simulink model "ASM_Traffic"  (R2026a)
settings: Solver=ode1  StartTime=SIM.tstart.v  StopTime=SIM.tend.v  FixedStep=SIM.StepSize.v
PostLoadFcn:
  | if any(exist('dsrtsu_mdlpostloadfcn', 'file') ~= 0), dsrtsu_mdlpostloadfcn('Execute', bdroot); end
  | try, asm_mdl_postloadfcn(bdroot, 'UpdateModel', 3600); catch, disp(lasterr); end,
InitFcn:
  | , if any(exist('rtifpga_mdlclblib', 'file') ~= 0), rtifpga_mdlclblib('Init', bdroot); end,
  | , if any(exist('dsmpb_private', 'file') ~= 0), dsmpb_private('dsmpb_mdlclblib', 'Init', bdroot); end,
model workspace (MAT data in the model file):
  asmReferencePath = [0 0.01 0.02 0.03 0.04 0.05 0.06 0.07 0.08 0.09 0.1 0.11 ... (350007 elements, 50001x7)]
  roadBounds : Simulink.Parameter (value not decoded)
  safetyAxes : Simulink.Parameter (value not decoded)
undefined symbols (not defined in the file): _to_, a0b2, ASM_BrakeHydraulics_DemoSystems, ASM_VehicleDynamics_DemoSystems, b98103fe8ad365046cd0, BrakeCircuit, controllerConfig, CPT, Crankshaft, DiscIntNeverNeededParam, dsmsi, FinalDriveAssembly, MDL, ModeSignals, mu, Pos_BrakePedal_Maneuver, rad, RefSignals, roadFamilyData, roadFamilyId, s_to_rpm, SIM, SoftECU, Suspension, Tire, Transmission
libraries: ASM_Traffic_lib x135, simulink x98, ASM_Utils_lib x77, ASM_VehicleDynamics_lib x70, ASM_Environment_lib x22, dsmpblib x20, dsmsilib x15, MDLD_Utils_lib x10, ASM_BrakeHydraulics_lib x3, sl_discontinuities x2
(part 38 of 65)

== system ASM_Traffic/Engine/Plant/UserInterface/DISP_Plant/Fuel_Consumption[L|100km]_ ==
  note: If v_Vehicle < v_Vehicle_LowLim, Then FuelConsumption = [L|h]
      | Else, FuelConsumption = [L|100km]
  v_Vehicle[km|h] : Inport
  Fuel_Consumption[l|h] : Inport  Port=2
  100 : Constant  Value=100
  999 : Constant  Value=999
  FuelConsumption : Terminator
  FuelConsumption[L|100km]_ : Product  Inputs=/**  SaturateOnIntegerOverflow=on  OutDataTypeStr=Inherit: Same as first input
  Sat_v_Vehicle[km|h] : Saturate  UpperLimit=inf  LowerLimit=eps
  Sw_FuelConsumption[L|100km] : MultiPortSwitch  DataPortOrder=Zero-based contiguous  Inputs=2  zeroidx=on  SaturateOnIntegerOverflow=off  InputSameDT=off
  Sw_[L|100km]2[L|h] : Switch  Criteria=u2 > Threshold  SaturateOnIntegerOverflow=off  InputSameDT=off
  v_Vehicle_LowLim[km|h] : simulink/Logic and Bit Operations/Compare To Constant  relop=>=  const=1  OutDataTypeStr=boolean
  Fuel_Consumption[L|100km] : Outport  VectorParamsAs1DForOutWhenUnconnected=off
  wires:
  999/1 -> Sw_FuelConsumption[L|100km]/2
  FuelConsumption[L|100km]_/1 -> Sw_FuelConsumption[L|100km]/3
  Sw_[L|100km]2[L|h]/1 -> FuelConsumption/1
  v_Vehicle_LowLim[km|h]/1 -> Sw_[L|100km]2[L|h]/2, Sw_FuelConsumption[L|100km]/1
  Sat_v_Vehicle[km|h]/1 -> FuelConsumption[L|100km]_/1
  100/1 -> FuelConsumption[L|100km]_/3
  Fuel_Consumption[l|h]/1 -> Sw_[L|100km]2[L|h]/3, FuelConsumption[L|100km]_/2
  v_Vehicle[km|h]/1 -> v_Vehicle_LowLim[km|h]/1, Sat_v_Vehicle[km|h]/1
  Sw_FuelConsumption[L|100km]/1 -> Sw_[L|100km]2[L|h]/1, Fuel_Consumption[L|100km]/1

== system ASM_Traffic/Engine/Plant/UserInterface/DISP_Plant/Fuel_Consumption[l|h] ==
  In1 : Inport
  Out1 : Outport  VectorParamsAs1DForOutWhenUnconnected=off
  wires:
  In1/1 -> Out1/1

== system ASM_Traffic/Engine/Plant/UserInterface/DISP_Plant/Fuel_Consumption_Total[l] ==
  In1 : Inport
  Out1 : Outport  VectorParamsAs1DForOutWhenUnconnected=off
  wires:
  In1/1 -> Out1/1

== system ASM_Traffic/Engine/Plant/UserInterface/DISP_Plant/T_Water[degC] ==
  In1 : Inport
  Out1 : Outport  VectorParamsAs1DForOutWhenUnconnected=off
  wires:
  In1/1 -> Out1/1

== system ASM_Traffic/Engine/Plant/UserInterface/DISP_Plant/Trq_Eff_Engine[Nm] ==
  In1 : Inport
  Out1 : Outport  VectorParamsAs1DForOutWhenUnconnected=off
  wires:
  In1/1 -> Out1/1

== system ASM_Traffic/Engine/Plant/UserInterface/DISP_Plant/Trq_Fric_Engine[Nm] ==
  In1 : Inport
  Out1 : Outport  VectorParamsAs1DForOutWhenUnconnected=off
  wires:
  In1/1 -> Out1/1

== system ASM_Traffic/Engine/Plant/UserInterface/DISP_Plant/Trq_Ind_Engine[Nm] ==
  In1 : Inport
  Out1 : Outport  VectorParamsAs1DForOutWhenUnconnected=off
  wires:
  In1/1 -> Out1/1

== system ASM_Traffic/Engine/Plant/UserInterface/DISP_Plant/b_e[g|kWh] ==
  In1 : Inport
  Out1 : Outport  VectorParamsAs1DForOutWhenUnconnected=off
  wires:
  In1/1 -> Out1/1

== system ASM_Traffic/Engine/Plant/UserInterface/DISP_Plant/eta_Eff_Engine[0_1] ==
  In1 : Inport
  Out1 : Outport  VectorParamsAs1DForOutWhenUnconnected=off
  wires:
  In1/1 -> Out1/1

== system ASM_Traffic/Engine/Plant/UserInterface/DISP_Plant/eta_Ind_Engine[0_1] ==
  In1 : Inport
  Out1 : Outport  VectorParamsAs1DForOutWhenUnconnected=off
  wires:
  In1/1 -> Out1/1

== system ASM_Traffic/Engine/Plant/UserInterface/DISP_Plant/eta_Mechanical_Engine[0_1] ==
  In1 : Inport
  Out1 : Outport  VectorParamsAs1DForOutWhenUnconnected=off
  wires:
  In1/1 -> Out1/1

== system ASM_Traffic/Engine/Plant/UserInterface/DISP_Plant/mdot_Fuel[g|h] ==
  In1 : Inport
  Out1 : Outport  VectorParamsAs1DForOutWhenUnconnected=off
  wires:
  In1/1 -> Out1/1

== system ASM_Traffic/Engine/SignalInterface/ASMSignalInterface/signal_structure/InfoBlock ==

== system ASM_Traffic/Environment/GroundTruth/PlantModel/Add_Time/Reset_Time ==
  Seconds_In[s] : Inport
  Add5 : Sum  Inputs=+-
  Constant4 : Constant  Value=86400
  Constant5 : Constant  Value=86400
  Divide2 : Product  Inputs=*/
  Divide3 : Product  Inputs=**
  Rounding Function3 : Rounding
  Seconds_Out[s] : Outport  VectorParamsAs1DForOutWhenUnconnected=off
  wires:
  Divide3/1 -> Add5/2
  Divide2/1 -> Rounding Function3/1
  Constant5/1 -> Divide3/2
  Add5/1 -> Seconds_Out[s]/1
  Seconds_In[s]/1 -> Add5/1, Divide2/1
  Constant4/1 -> Divide2/2
  Rounding Function3/1 -> Divide3/1

== system ASM_Traffic/Environment/GroundTruth/PlantModel/GroundTruth_Data_Access/GroundTruth_Access_Laneboundaries ==
  Enable[0Off|1On] : Inport
  OSI_GT_Data : Inport  Port=2
  Enable : EnablePort
  asm_trf_osi_access_laneboundaries : S-Function  FunctionName=asm_trf_osi_access_laneboundaries  Parameters=10,15  SFunctionDeploymentMode=off  EnableBusSupport=off
  Num_Laneboundaries[] : Outport  VectorParamsAs1DForOutWhenUnconnected=off
  Laneboundary_ID[] : Outport  Port=2  VectorParamsAs1DForOutWhenUnconnected=off
  Laneboundary_Type[] : Outport  Port=3  VectorParamsAs1DForOutWhenUnconnected=off
  Laneboundary_Color[] : Outport  Port=4  VectorParamsAs1DForOutWhenUnconnected=off
  Num_Laneboundary_Points[] : Outport  Port=5  VectorParamsAs1DForOutWhenUnconnected=off
  Laneboundary_Point_Width[m] : Outport  Port=6  VectorParamsAs1DForOutWhenUnconnected=off
  Laneboundary_Point_Height[m] : Outport  Port=7  VectorParamsAs1DForOutWhenUnconnected=off
  Laneboundary_Point_Pos_x[m] : Outport  Port=8  VectorParamsAs1DForOutWhenUnconnected=off
  Laneboundary_Point_Pos_y[m] : Outport  Port=9  VectorParamsAs1DForOutWhenUnconnected=off
  Laneboundary_Point_Pos_z[m] : Outport  Port=10  VectorParamsAs1DForOutWhenUnconnected=off
  Laneboundary_Point_Dash[] : Outport  Port=11  VectorParamsAs1DForOutWhenUnconnected=off
  wires:
  asm_trf_osi_access_laneboundaries/11 -> Laneboundary_Point_Dash[]/1
  asm_trf_osi_access_laneboundaries/10 -> Laneboundary_Point_Pos_z[m]/1
  asm_trf_osi_access_laneboundaries/9 -> Laneboundary_Point_Pos_y[m]/1
  asm_trf_osi_access_laneboundaries/8 -> Laneboundary_Point_Pos_x[m]/1
  asm_trf_osi_access_laneboundaries/7 -> Laneboundary_Point_Height[m]/1
  asm_trf_osi_access_laneboundaries/6 -> Laneboundary_Point_Width[m]/1
  asm_trf_osi_access_laneboundaries/5 -> Num_Laneboundary_Points[]/1
  asm_trf_osi_access_laneboundaries/4 -> Laneboundary_Color[]/1
  asm_trf_osi_access_laneboundaries/3 -> Laneboundary_Type[]/1
  asm_trf_osi_access_laneboundaries/2 -> Laneboundary_ID[]/1
  asm_trf_osi_access_laneboundaries/1 -> Num_Laneboundaries[]/1
  OSI_GT_Data/1 -> asm_trf_osi_access_laneboundaries/2
  Enable[0Off|1On]/1 -> asm_trf_osi_access_laneboundaries/1

== system ASM_Traffic/Environment/GroundTruth/PlantModel/GroundTruth_Data_Access/GroundTruth_Access_Lanes ==
  Enable[0Off|1On] : Inport
  OSI_GT_Data : Inport  Port=2
  asm_trf_osi_access_lanes : S-Function  FunctionName=asm_trf_osi_access_lanes  Parameters=20,10,10  SFunctionDeploymentMode=off  EnableBusSupport=off
  Num_Lanes[] : Outport  VectorParamsAs1DForOutWhenUnconnected=off
  Lane_ID[] : Outport  Port=2  VectorParamsAs1DForOutWhenUnconnected=off
  Lane_Type[] : Outport  Port=3  VectorParamsAs1DForOutWhenUnconnected=off
  Is_Host_Vehicle_Lane[0|1] : Outport  Port=4  VectorParamsAs1DForOutWhenUnconnected=off
  Num_Left_Adjacent_Lanes[] : Outport  Port=5  VectorParamsAs1DForOutWhenUnconnected=off
  Left_Adjacent_Lane_ID[m] : Outport  Port=6  VectorParamsAs1DForOutWhenUnconnected=off
  Num_Right_Adjacent_Lanes[] : Outport  Port=7  VectorParamsAs1DForOutWhenUnconnected=off
  Right_Adjacent_Lane_ID[m] : Outport  Port=8  VectorParamsAs1DForOutWhenUnconnected=off
  Num_Lane_Pairings[] : Outport  Port=9  VectorParamsAs1DForOutWhenUnconnected=off
  Successor_Lane_ID[] : Outport  Port=10  VectorParamsAs1DForOutWhenUnconnected=off
  Antecessor_Lane_ID[] : Outport  Port=11  VectorParamsAs1DForOutWhenUnconnected=off
  Num_Left_Laneboundaries[] : Outport  Port=12  VectorParamsAs1DForOutWhenUnconnected=off
  Left_Laneboundary_ID[] : Outport  Port=13  VectorParamsAs1DForOutWhenUnconnected=off
  Num_Right_Laneboundaries[] : Outport  Port=14  VectorParamsAs1DForOutWhenUnconnected=off
  Right_Laneboundary_ID[] : Outport  Port=15  VectorParamsAs1DForOutWhenUnconnected=off
  Num_Free_Laneboundaries[] : Outport  Port=16  VectorParamsAs1DForOutWhenUnconnected=off
  Free_Laneboundary_ID[] : Outport  Port=17  VectorParamsAs1DForOutWhenUnconnected=off
  wires:
  Enable[0Off|1On]/1 -> asm_trf_osi_access_lanes/1
  OSI_GT_Data/1 -> asm_trf_osi_access_lanes/2
  asm_trf_osi_access_lanes/1 -> Num_Lanes[]/1
  asm_trf_osi_access_lanes/2 -> Lane_ID[]/1
  asm_trf_osi_access_lanes/3 -> Lane_Type[]/1
  asm_trf_osi_access_lanes/4 -> Is_Host_Vehicle_Lane[0|1]/1
  asm_trf_osi_access_lanes/5 -> Num_Left_Adjacent_Lanes[]/1
  asm_trf_osi_access_lanes/6 -> Left_Adjacent_Lane_ID[m]/1
  asm_trf_osi_access_lanes/7 -> Num_Right_Adjacent_Lanes[]/1
  asm_trf_osi_access_lanes/8 -> Right_Adjacent_Lane_ID[m]/1
  asm_trf_osi_access_lanes/9 -> Num_Lane_Pairings[]/1
  asm_trf_osi_access_lanes/10 -> Successor_Lane_ID[]/1
  asm_trf_osi_access_lanes/11 -> Antecessor_Lane_ID[]/1
  asm_trf_osi_access_lanes/12 -> Num_Left_Laneboundaries[]/1
  asm_trf_osi_access_lanes/13 -> Left_Laneboundary_ID[]/1
  asm_trf_osi_access_lanes/14 -> Num_Right_Laneboundaries[]/1
  asm_trf_osi_access_lanes/15 -> Right_Laneboundary_ID[]/1
  asm_trf_osi_access_lanes/16 -> Num_Free_Laneboundaries[]/1
  asm_trf_osi_access_lanes/17 -> Free_Laneboundary_ID[]/1

== system ASM_Traffic/Environment/GroundTruth/PlantModel/GroundTruth_Data_Access/GroundTruth_Access_MovingObjects ==
  Enable[0Off|1On] : Inport
  Filter_MovObj_In_GT_Area[0Off|1On] : Inport  Port=2
  MovObj_Idx[] : Inport  Port=3
  OSI_GT_Data : Inport  Port=4
  asm_trf_osi_access_mov_obj : S-Function  FunctionName=asm_trf_osi_access_mov_obj  Parameters=10  SFunctionDeploymentMode=off  EnableBusSupport=off
  Num_MovObj[] : Outport  VectorParamsAs1DForOutWhenUnconnected=off
  Num_MovObj_in_GT_Area[] : Outport  Port=2  VectorParamsAs1DForOutWhenUnconnected=off
  Flag_MovObj_in_GT_Area[] : Outport  Port=3  VectorParamsAs1DForOutWhenUnconnected=off
  MovObj_Type[] : Outport  Port=4  VectorParamsAs1DForOutWhenUnconnected=off
  MovObj_Vehicle_Type[] : Outport  Port=5  VectorParamsAs1DForOutWhenUnconnected=off
  MovObj_ID[] : Outport  Port=6  VectorParamsAs1DForOutWhenUnconnected=off
  MovObj_Driver_ID[] : Outport  Port=7  VectorParamsAs1DForOutWhenUnconnected=off
  Flag_MovObj_HasTrailer[] : Outport  Port=8  VectorParamsAs1DForOutWhenUnconnected=off
  MovObj_Trailer_ID[] : Outport  Port=9  VectorParamsAs1DForOutWhenUnconnected=off
  MovObj_Position_x[m] : Outport  Port=10  VectorParamsAs1DForOutWhenUnconnected=off
  MovObj_Position_y[m] : Outport  Port=11  VectorParamsAs1DForOutWhenUnconnected=off
  MovObj_Position_z[m] : Outport  Port=12  VectorParamsAs1DForOutWhenUnconnected=off
  MovObj_Velocity_x[km|h] : Outport  Port=13  VectorParamsAs1DForOutWhenUnconnected=off
  MovObj_Velocity_y[km|h] : Outport  Port=14  VectorParamsAs1DForOutWhenUnconnected=off
  MovObj_Velocity_z[km|h] : Outport  Port=15  VectorParamsAs1DForOutWhenUnconnected=off
  MovObj_Acceleration_x[m|s2] : Outport  Port=16  VectorParamsAs1DForOutWhenUnconnected=off
  MovObj_Acceleration_y[m|s2] : Outport  Port=17  VectorParamsAs1DForOutWhenUnconnected=off
  MovObj_Acceleration_z[m|s2] : Outport  Port=18  VectorParamsAs1DForOutWhenUnconnected=off
  MovObj_Orientation_x[deg] : Outport  Port=19  VectorParamsAs1DForOutWhenUnconnected=off
  MovObj_Orientation_y[deg] : Outport  Port=20  VectorParamsAs1DForOutWhenUnconnected=off
  MovObj_Orientation_z[deg] : Outport  Port=21  VectorParamsAs1DForOutWhenUnconnected=off
  MovObj_OrientationRate_x[deg|s] : Outport  Port=22  VectorParamsAs1DForOutWhenUnconnected=off
  MovObj_OrientationRate_y[deg|s] : Outport  Port=23  VectorParamsAs1DForOutWhenUnconnected=off
  MovObj_OrientationRate_z[deg|s] : Outport  Port=24  VectorParamsAs1DForOutWhenUnconnected=off
  MovObj_OrientationAcceleration_x[deg|s2] : Outport  Port=25  VectorParamsAs1DForOutWhenUnconnected=off
  MovObj_OrientationAcceleration_y[deg|s2] : Outport  Port=26  VectorParamsAs1DForOutWhenUnconnected=off
  MovObj_OrientationAcceleration_z[deg|s2] : Outport  Port=27  VectorParamsAs1DForOutWhenUnconnected=off
  MovObj_Length[m] : Outport  Port=28  VectorParamsAs1DForOutWhenUnconnected=off
  MovObj_Width[m] : Outport  Port=29  VectorParamsAs1DForOutWhenUnconnected=off
  MovObj_Height[m] : Outport  Port=30  VectorParamsAs1DForOutWhenUnconnected=off
  MovObj_PolyPts_x[m] : Outport  Port=31  VectorParamsAs1DForOutWhenUnconnected=off
  MovObj_PolyPts_y[m] : Outport  Port=32  VectorParamsAs1DForOutWhenUnconnected=off
  MovObj_BBCenter_To_Front_x[m] : Outport  Port=33  VectorParamsAs1DForOutWhenUnconnected=off
  MovObj_BBCenter_To_Front_y[m] : Outport  Port=34  VectorParamsAs1DForOutWhenUnconnected=off
  MovObj_BBCenter_To_Front_z[m] : Outport  Port=35  VectorParamsAs1DForOutWhenUnconnected=off
  MovObj_BBCenter_To_Rear_x[m] : Outport  Port=36  VectorParamsAs1DForOutWhenUnconnected=off
  MovObj_BBCenter_To_Rear_y[m] : Outport  Port=37  VectorParamsAs1DForOutWhenUnconnected=off
  MovObj_BBCenter_To_Rear_z[m] : Outport  Port=38  VectorParamsAs1DForOutWhenUnconnected=off
  MovObj_Num_Wheels[] : Outport  Port=39  VectorParamsAs1DForOutWhenUnconnected=off
  MovObj_GroundClearance[m] : Outport  Port=40  VectorParamsAs1DForOutWhenUnconnected=off
  MovObj_WheelRadius[m] : Outport  Port=41  VectorParamsAs1DForOutWhenUnconnected=off
  MovObj_Lights[] : Outport  Port=42  VectorParamsAs1DForOutWhenUnconnected=off
  MovObj_NumLanes[] : Outport  Port=43  VectorParamsAs1DForOutWhenUnconnected=off
  MovObj_Lane_ID_1[] : Outport  Port=44  VectorParamsAs1DForOutWhenUnconnected=off
  MovObj_Lane_ID_2[] : Outport  Port=45  VectorParamsAs1DForOutWhenUnconnected=off
  wires:
  asm_trf_osi_access_mov_obj/45 -> MovObj_Lane_ID_2[]/1
  asm_trf_osi_access_mov_obj/44 -> MovObj_Lane_ID_1[]/1
  asm_trf_osi_access_mov_obj/43 -> MovObj_NumLanes[]/1
  asm_trf_osi_access_mov_obj/42 -> MovObj_Lights[]/1
  asm_trf_osi_access_mov_obj/41 -> MovObj_WheelRadius[m]/1
  asm_trf_osi_access_mov_obj/40 -> MovObj_GroundClearance[m]/1
  asm_trf_osi_access_mov_obj/39 -> MovObj_Num_Wheels[]/1
  asm_trf_osi_access_mov_obj/38 -> MovObj_BBCenter_To_Rear_z[m]/1
  asm_trf_osi_access_mov_obj/37 -> MovObj_BBCenter_To_Rear_y[m]/1
  asm_trf_osi_access_mov_obj/36 -> MovObj_BBCenter_To_Rear_x[m]/1
  asm_trf_osi_access_mov_obj/34 -> MovObj_BBCenter_To_Front_y[m]/1
  asm_trf_osi_access_mov_obj/35 -> MovObj_BBCenter_To_Front_z[m]/1
  asm_trf_osi_access_mov_obj/33 -> MovObj_BBCenter_To_Front_x[m]/1
  asm_trf_osi_access_mov_obj/32 -> MovObj_PolyPts_y[m]/1
  asm_trf_osi_access_mov_obj/31 -> MovObj_PolyPts_x[m]/1
  asm_trf_osi_access_mov_obj/30 -> MovObj_Height[m]/1
  asm_trf_osi_access_mov_obj/29 -> MovObj_Width[m]/1
  asm_trf_osi_access_mov_obj/28 -> MovObj_Length[m]/1
  asm_trf_osi_access_mov_obj/27 -> MovObj_OrientationAcceleration_z[deg|s2]/1
  asm_trf_osi_access_mov_obj/26 -> MovObj_OrientationAcceleration_y[deg|s2]/1
  asm_trf_osi_access_mov_obj/25 -> MovObj_OrientationAcceleration_x[deg|s2]/1
  asm_trf_osi_access_mov_obj/24 -> MovObj_OrientationRate_z[deg|s]/1
  asm_trf_osi_access_mov_obj/23 -> MovObj_OrientationRate_y[deg|s]/1
  asm_trf_osi_access_mov_obj/22 -> MovObj_OrientationRate_x[deg|s]/1
  asm_trf_osi_access_mov_obj/21 -> MovObj_Orientation_z[deg]/1
  asm_trf_osi_access_mov_obj/20 -> MovObj_Orientation_y[deg]/1
  asm_trf_osi_access_mov_obj/19 -> MovObj_Orientation_x[deg]/1
  asm_trf_osi_access_mov_obj/18 -> MovObj_Acceleration_z[m|s2]/1
  asm_trf_osi_access_mov_obj/17 -> MovObj_Acceleration_y[m|s2]/1
  asm_trf_osi_access_mov_obj/16 -> MovObj_Acceleration_x[m|s2]/1
  asm_trf_osi_access_mov_obj/15 -> MovObj_Velocity_z[km|h]/1
  asm_trf_osi_access_mov_obj/14 -> MovObj_Velocity_y[km|h]/1
  asm_trf_osi_access_mov_obj/13 -> MovObj_Velocity_x[km|h]/1
  asm_trf_osi_access_mov_obj/12 -> MovObj_Position_z[m]/1
  asm_trf_osi_access_mov_obj/11 -> MovObj_Position_y[m]/1
  asm_trf_osi_access_mov_obj/10 -> MovObj_Position_x[m]/1
  asm_trf_osi_access_mov_obj/9 -> MovObj_Trailer_ID[]/1
  asm_trf_osi_access_mov_obj/8 -> Flag_MovObj_HasTrailer[]/1
  asm_trf_osi_access_mov_obj/7 -> MovObj_Driver_ID[]/1
  asm_trf_osi_access_mov_obj/6 -> MovObj_ID[]/1
  asm_trf_osi_access_mov_obj/5 -> MovObj_Vehicle_Type[]/1
  asm_trf_osi_access_mov_obj/4 -> MovObj_Type[]/1
  asm_trf_osi_access_mov_obj/3 -> Flag_MovObj_in_GT_Area[]/1
  asm_trf_osi_access_mov_obj/2 -> Num_MovObj_in_GT_Area[]/1
  asm_trf_osi_access_mov_obj/1 -> Num_MovObj[]/1
  OSI_GT_Data/1 -> asm_trf_osi_access_mov_obj/4
  MovObj_Idx[]/1 -> asm_trf_osi_access_mov_obj/3
  Filter_MovObj_In_GT_Area[0Off|1On]/1 -> asm_trf_osi_access_mov_obj/2
  Enable[0Off|1On]/1 -> asm_trf_osi_access_mov_obj/1

== system ASM_Traffic/Environment/GroundTruth/PlantModel/GroundTruth_Data_Access/GroundTruth_Access_StationaryObjects ==
  Enable[0Off|1On] : Inport
  Filter_StatObj_In_GT_Area[0Off|1On] : Inport  Port=2
  StatObj_Idx[] : Inport  Port=3
  OSI_GT_Data : Inport  Port=4
  asm_trf_osi_access_stat_obj : S-Function  FunctionName=asm_trf_osi_access_stat_obj  Parameters=10  SFunctionDeploymentMode=off  EnableBusSupport=off
  Num_StatObj[] : Outport  VectorParamsAs1DForOutWhenUnconnected=off
  Num_StatObj_in_GT_Area[] : Outport  Port=2  VectorParamsAs1DForOutWhenUnconnected=off
  Flag_StatObj_in_GT_Area[] : Outport  Port=3  VectorParamsAs1DForOutWhenUnconnected=off
  StatObj_Type[] : Outport  Port=4  VectorParamsAs1DForOutWhenUnconnected=off
  StatObj_ID[] : Outport  Port=5  VectorParamsAs1DForOutWhenUnconnected=off
  StatObj_Material[] : Outport  Port=6  VectorParamsAs1DForOutWhenUnconnected=off
  StatObj_Density[] : Outport  Port=7  VectorParamsAs1DForOutWhenUnconnected=off
  StatObj_Color[] : Outport  Port=8  VectorParamsAs1DForOutWhenUnconnected=off
  StatObj_Position_x[m] : Outport  Port=9  VectorParamsAs1DForOutWhenUnconnected=off
  StatObj_Position_y[m] : Outport  Port=10  VectorParamsAs1DForOutWhenUnconnected=off
  StatObj_Position_z[m] : Outport  Port=11  VectorParamsAs1DForOutWhenUnconnected=off
  StatObj_Orientation_x[deg] : Outport  Port=12  VectorParamsAs1DForOutWhenUnconnected=off
  StatObj_Orientation_y[deg] : Outport  Port=13  VectorParamsAs1DForOutWhenUnconnected=off
  StatObj_Orientation_z[deg] : Outport  Port=14  VectorParamsAs1DForOutWhenUnconnected=off
  StatObj_Length[m] : Outport  Port=15  VectorParamsAs1DForOutWhenUnconnected=off
  StatObj_Width[m] : Outport  Port=16  VectorParamsAs1DForOutWhenUnconnected=off
  StatObj_Height[m] : Outport  Port=17  VectorParamsAs1DForOutWhenUnconnected=off
  StatObj_PolyPts_x[m] : Outport  Port=18  VectorParamsAs1DForOutWhenUnconnected=off
  StatObj_PolyPts_y[m] : Outport  Port=19  VectorParamsAs1DForOutWhenUnconnected=off
  wires:
  Enable[0Off|1On]/1 -> asm_trf_osi_access_stat_obj/1
  Filter_StatObj_In_GT_Area[0Off|1On]/1 -> asm_trf_osi_access_stat_obj/2
  StatObj_Idx[]/1 -> asm_trf_osi_access_stat_obj/3
  OSI_GT_Data/1 -> asm_trf_osi_access_stat_obj/4
  asm_trf_osi_access_stat_obj/1 -> Num_StatObj[]/1
  asm_trf_osi_access_stat_obj/2 -> Num_StatObj_in_GT_Area[]/1
  asm_trf_osi_access_stat_obj/3 -> Flag_StatObj_in_GT_Area[]/1
  asm_trf_osi_access_stat_obj/4 -> StatObj_Type[]/1
  asm_trf_osi_access_stat_obj/5 -> StatObj_ID[]/1
  asm_trf_osi_access_stat_obj/6 -> StatObj_Material[]/1
  asm_trf_osi_access_stat_obj/7 -> StatObj_Density[]/1
  asm_trf_osi_access_stat_obj/8 -> StatObj_Color[]/1
  asm_trf_osi_access_stat_obj/9 -> StatObj_Position_x[m]/1
  asm_trf_osi_access_stat_obj/10 -> StatObj_Position_y[m]/1
  asm_trf_osi_access_stat_obj/11 -> StatObj_Position_z[m]/1
  asm_trf_osi_access_stat_obj/12 -> StatObj_Orientation_x[deg]/1
  asm_trf_osi_access_stat_obj/13 -> StatObj_Orientation_y[deg]/1
  asm_trf_osi_access_stat_obj/14 -> StatObj_Orientation_z[deg]/1
  asm_trf_osi_access_stat_obj/15 -> StatObj_Length[m]/1
  asm_trf_osi_access_stat_obj/16 -> StatObj_Width[m]/1
  asm_trf_osi_access_stat_obj/17 -> StatObj_Height[m]/1
  asm_trf_osi_access_stat_obj/18 -> StatObj_PolyPts_x[m]/1
  asm_trf_osi_access_stat_obj/19 -> StatObj_PolyPts_y[m]/1

== system ASM_Traffic/Environment/GroundTruth/PlantModel/GroundTruth_Data_Access/GroundTruth_Access_TrafficLights ==
  Enable[0Off|1On] : Inport
  Filter_TrfLight_In_GT_Area[0Off|1On] : Inport  Port=2
  TrfLight_Idx[] : Inport  Port=3
  OSI_GT_Data : Inport  Port=4
  asm_trf_osi_access_trf_lights : S-Function  FunctionName=asm_trf_osi_access_trf_lights  Parameters=10  SFunctionDeploymentMode=off  EnableBusSupport=off
  Num_TrfLights[] : Outport  VectorParamsAs1DForOutWhenUnconnected=off
  Num_TrfLights_in_GT_Area[] : Outport  Port=2  VectorParamsAs1DForOutWhenUnconnected=off
  Flag_TrfLight_in_GT_Area[] : Outport  Port=3  VectorParamsAs1DForOutWhenUnconnected=off
  TrfLight_ID[] : Outport  Port=4  VectorParamsAs1DForOutWhenUnconnected=off
  TrfLight_Mode[] : Outport  Port=5  VectorParamsAs1DForOutWhenUnconnected=off
  TrfLight_Color[] : Outport  Port=6  VectorParamsAs1DForOutWhenUnconnected=off
  TrfLight_Icon[] : Outport  Port=7  VectorParamsAs1DForOutWhenUnconnected=off
  TrfLight_Counter[] : Outport  Port=8  VectorParamsAs1DForOutWhenUnconnected=off
  TrfLight_Position_x[m] : Outport  Port=9  VectorParamsAs1DForOutWhenUnconnected=off
  TrfLight_Position_y[m] : Outport  Port=10  VectorParamsAs1DForOutWhenUnconnected=off
  TrfLight_Position_z[m] : Outport  Port=11  VectorParamsAs1DForOutWhenUnconnected=off
  TrfLight_Orientation_x[deg] : Outport  Port=12  VectorParamsAs1DForOutWhenUnconnected=off
  TrfLight_Orientation_y[deg] : Outport  Port=13  VectorParamsAs1DForOutWhenUnconnected=off
  TrfLight_Orientation_z[deg] : Outport  Port=14  VectorParamsAs1DForOutWhenUnconnected=off
  TrfLight_Length[m] : Outport  Port=15  VectorParamsAs1DForOutWhenUnconnected=off
  TrfLight_Width[m] : Outport  Port=16  VectorParamsAs1DForOutWhenUnconnected=off
  TrfLight_Height[m] : Outport  Port=17  VectorParamsAs1DForOutWhenUnconnected=off
  TrfLight_PolyPts_x[m] : Outport  Port=18  VectorParamsAs1DForOutWhenUnconnected=off
  TrfLight_PolyPts_y[m] : Outport  Port=19  VectorParamsAs1DForOutWhenUnconnected=off
  Num_Assigned_Lanes[] : Outport  Port=20  VectorParamsAs1DForOutWhenUnconnected=off
  Assigned_Lane_ID[] : Outport  Port=21  VectorParamsAs1DForOutWhenUnconnected=off
  wires:
  asm_trf_osi_access_trf_lights/19 -> TrfLight_Height[m]/1
  asm_trf_osi_access_trf_lights/18 -> TrfLight_Width[m]/1
  asm_trf_osi_access_trf_lights/17 -> TrfLight_Length[m]/1
  asm_trf_osi_access_trf_lights/16 -> TrfLight_Orientation_z[deg]/1
  asm_trf_osi_access_trf_lights/15 -> TrfLight_Orientation_y[deg]/1
  asm_trf_osi_access_trf_lights/14 -> TrfLight_Orientation_x[deg]/1
  asm_trf_osi_access_trf_lights/13 -> TrfLight_Position_z[m]/1
  asm_trf_osi_access_trf_lights/12 -> TrfLight_Position_y[m]/1
  asm_trf_osi_access_trf_lights/11 -> TrfLight_Position_x[m]/1
  asm_trf_osi_access_trf_lights/10 -> Assigned_Lane_ID[]/1
  asm_trf_osi_access_trf_lights/9 -> Num_Assigned_Lanes[]/1
  asm_trf_osi_access_trf_lights/8 -> TrfLight_Counter[]/1
  asm_trf_osi_access_trf_lights/7 -> TrfLight_Icon[]/1
  asm_trf_osi_access_trf_lights/6 -> TrfLight_Color[]/1
  asm_trf_osi_access_trf_lights/5 -> TrfLight_Mode[]/1
  asm_trf_osi_access_trf_lights/4 -> TrfLight_ID[]/1
  asm_trf_osi_access_trf_lights/3 -> Flag_TrfLight_in_GT_Area[]/1
  asm_trf_osi_access_trf_lights/2 -> Num_TrfLights_in_GT_Area[]/1
  asm_trf_osi_access_trf_lights/1 -> Num_TrfLights[]/1
  OSI_GT_Data/1 -> asm_trf_osi_access_trf_lights/4
  TrfLight_Idx[]/1 -> asm_trf_osi_access_trf_lights/3
  Filter_TrfLight_In_GT_Area[0Off|1On]/1 -> asm_trf_osi_access_trf_lights/2
  Enable[0Off|1On]/1 -> asm_trf_osi_access_trf_lights/1
  asm_trf_osi_access_trf_lights/20 -> TrfLight_PolyPts_x[m]/1
  asm_trf_osi_access_trf_lights/21 -> TrfLight_PolyPts_y[m]/1

== system ASM_Traffic/Environment/GroundTruth/PlantModel/GroundTruth_Data_Access/GroundTruth_Access_TrafficSigns ==
  Enable[0Off|1On] : Inport
  Filter_TrfSigns_In_GT_Area[0Off|1On] : Inport  Port=2
  TrfSign_Idx[] : Inport  Port=3
  OSI_GT_Data : Inport  Port=4
  asm_trf_osi_access_trf_signs : S-Function  FunctionName=asm_trf_osi_access_trf_signs  Parameters=10,2  SFunctionDeploymentMode=off  EnableBusSupport=off
  Num_TrfSigns[] : Outport  VectorParamsAs1DForOutWhenUnconnected=off
  Num_TrfSigns_in_GT_Area[] : Outport  Port=2  VectorParamsAs1DForOutWhenUnconnected=off
  Flag_TrfSign_in_GT_Area[] : Outport  Port=3  VectorParamsAs1DForOutWhenUnconnected=off
  Num_SupplementarySigns[] : Outport  Port=4  VectorParamsAs1DForOutWhenUnconnected=off
  TrfSign_ID[] : Outport  Port=5  VectorParamsAs1DForOutWhenUnconnected=off
  TrfSign_Type[] : Outport  Port=6  VectorParamsAs1DForOutWhenUnconnected=off
  TrfSign_VerticallyMirrored[] : Outport  Port=7  VectorParamsAs1DForOutWhenUnconnected=off
  TrfSign_DirectionScope[] : Outport  Port=8  VectorParamsAs1DForOutWhenUnconnected=off
  TrfSign_Value_Unit[] : Outport  Port=9  VectorParamsAs1DForOutWhenUnconnected=off
  TrfSign_Num_AssignedLanes[] : Outport  Port=10  VectorParamsAs1DForOutWhenUnconnected=off
  TrfSign_AssignedLanes[m] : Outport  Port=11  VectorParamsAs1DForOutWhenUnconnected=off
  TrfSign_Position_x[m] : Outport  Port=12  VectorParamsAs1DForOutWhenUnconnected=off
  TrfSign_Position_y[m] : Outport  Port=13  VectorParamsAs1DForOutWhenUnconnected=off
  TrfSign_Position_z[m] : Outport  Port=14  VectorParamsAs1DForOutWhenUnconnected=off
  TrfSign_Orientation_x[deg] : Outport  Port=15  VectorParamsAs1DForOutWhenUnconnected=off
  TrfSign_Orientation_y[deg] : Outport  Port=16  VectorParamsAs1DForOutWhenUnconnected=off
  TrfSign_Orientation_z[deg] : Outport  Port=17  VectorParamsAs1DForOutWhenUnconnected=off
  TrfSign_Length[m] : Outport  Port=18  VectorParamsAs1DForOutWhenUnconnected=off
  TrfSign_Width[m] : Outport  Port=19  VectorParamsAs1DForOutWhenUnconnected=off
  TrfSign_Variability[] : Outport  Port=20  VectorParamsAs1DForOutWhenUnconnected=off
  TrfSign_Value[] : Outport  Port=21  VectorParamsAs1DForOutWhenUnconnected=off
  TrfSign_Height[m] : Outport  Port=22  VectorParamsAs1DForOutWhenUnconnected=off
  TrfSign_PolyPts_x[m] : Outport  Port=23  VectorParamsAs1DForOutWhenUnconnected=off
  TrfSign_PolyPts_y[m] : Outport  Port=24  VectorParamsAs1DForOutWhenUnconnected=off
  SupplementarySign_Type[] : Outport  Port=25  VectorParamsAs1DForOutWhenUnconnected=off
  SupplementarySign_Actor[] : Outport  Port=26  VectorParamsAs1DForOutWhenUnconnected=off
  SupplementarySign_Variability[] : Outport  Port=27  VectorParamsAs1DForOutWhenUnconnected=off
  SupplementarySign_Value[] : Outport  Port=28  VectorParamsAs1DForOutWhenUnconnected=off
  SupplementarySign_Value_Unit[] : Outport  Port=29  VectorParamsAs1DForOutWhenUnconnected=off
  SupplementarySign_Num_AssignedLanes[] : Outport  Port=30  VectorParamsAs1DForOutWhenUnconnected=off
  SupplementarySign_Num_DirectionArrows[] : Outport  Port=31  VectorParamsAs1DForOutWhenUnconnected=off
  SupplementarySign_DirectionArrow_1[] : Outport  Port=32  VectorParamsAs1DForOutWhenUnconnected=off
  SupplementarySign_DirectionArrow_2[] : Outport  Port=33  VectorParamsAs1DForOutWhenUnconnected=off
  wires:
  asm_trf_osi_access_trf_signs/21 -> TrfSign_Width[m]/1
  asm_trf_osi_access_trf_signs/20 -> TrfSign_Length[m]/1
  Enable[0Off|1On]/1 -> asm_trf_osi_access_trf_signs/1
  Filter_TrfSigns_In_GT_Area[0Off|1On]/1 -> asm_trf_osi_access_trf_signs/2
  TrfSign_Idx[]/1 -> asm_trf_osi_access_trf_signs/3
  OSI_GT_Data/1 -> asm_trf_osi_access_trf_signs/4
  asm_trf_osi_access_trf_signs/1 -> Num_TrfSigns[]/1
  asm_trf_osi_access_trf_signs/2 -> Num_TrfSigns_in_GT_Area[]/1
  asm_trf_osi_access_trf_signs/3 -> Flag_TrfSign_in_GT_Area[]/1
  asm_trf_osi_access_trf_signs/4 -> Num_SupplementarySigns[]/1
  asm_trf_osi_access_trf_signs/5 -> TrfSign_ID[]/1
  asm_trf_osi_access_trf_signs/6 -> TrfSign_Type[]/1
  asm_trf_osi_access_trf_signs/7 -> TrfSign_VerticallyMirrored[]/1
  asm_trf_osi_access_trf_signs/8 -> TrfSign_DirectionScope[]/1
  asm_trf_osi_access_trf_signs/9 -> TrfSign_Variability[]/1
  asm_trf_osi_access_trf_signs/10 -> TrfSign_Value[]/1
  asm_trf_osi_access_trf_signs/11 -> TrfSign_Value_Unit[]/1
  asm_trf_osi_access_trf_signs/12 -> TrfSign_Num_AssignedLanes[]/1
  asm_trf_osi_access_trf_signs/13 -> TrfSign_AssignedLanes[m]/1
  asm_trf_osi_access_trf_signs/14 -> TrfSign_Position_x[m]/1
  asm_trf_osi_access_trf_signs/15 -> TrfSign_Position_y[m]/1
  asm_trf_osi_access_trf_signs/16 -> TrfSign_Position_z[m]/1
  asm_trf_osi_access_trf_signs/17 -> TrfSign_Orientation_x[deg]/1
  asm_trf_osi_access_trf_signs/18 -> TrfSign_Orientation_y[deg]/1
  asm_trf_osi_access_trf_signs/19 -> TrfSign_Orientation_z[deg]/1
  asm_trf_osi_access_trf_signs/22 -> TrfSign_Height[m]/1
  asm_trf_osi_access_trf_signs/23 -> TrfSign_PolyPts_x[m]/1
  asm_trf_osi_access_trf_signs/24 -> TrfSign_PolyPts_y[m]/1
  asm_trf_osi_access_trf_signs/25 -> SupplementarySign_Type[]/1
  asm_trf_osi_access_trf_signs/26 -> SupplementarySign_Actor[]/1
  asm_trf_osi_access_trf_signs/27 -> SupplementarySign_Variability[]/1
  asm_trf_osi_access_trf_signs/28 -> SupplementarySign_Value[]/1
  asm_trf_osi_access_trf_signs/29 -> SupplementarySign_Value_Unit[]/1
  asm_trf_osi_access_trf_signs/30 -> SupplementarySign_Num_AssignedLanes[]/1
  asm_trf_osi_access_trf_signs/31 -> SupplementarySign_Num_DirectionArrows[]/1
  asm_trf_osi_access_trf_signs/32 -> SupplementarySign_DirectionArrow_1[]/1
  asm_trf_osi_access_trf_signs/33 -> SupplementarySign_DirectionArrow_2[]/1

== system ASM_Traffic/Environment/GroundTruth/PlantModel/HostVehicle_Data_Access/HostVehicle_Data_Access ==
  Enable[0Off|1On] : Inport
  OSI_HV_Data : Inport  Port=2
  asm_trf_osi_access_host_vehicle_data : S-Function  FunctionName=asm_trf_osi_access_host_vehicle_data  Parameters=2,6  SFunctionDeploymentMode=off  EnableBusSupport=off
  Time_Stamp_Seconds[s] : Outport  VectorParamsAs1DForOutWhenUnconnected=off
  Time_Stamp_Nanos[ns] : Outport  Port=2  VectorParamsAs1DForOutWhenUnconnected=off
  HV_ID[] : Outport  Port=3  VectorParamsAs1DForOutWhenUnconnected=off
  HV_Pos_BrakePedal[0_1] : Outport  Port=4  VectorParamsAs1DForOutWhenUnconnected=off
  HV_Position_BB[x;y;z][m] : Outport  Port=5  VectorParamsAs1DForOutWhenUnconnected=off
  HV_Velocity_BB[x;y;z][m|s] : Outport  Port=6  VectorParamsAs1DForOutWhenUnconnected=off
  HV_Acceleration_BB[x;y;z][m|s2] : Outport  Port=7  VectorParamsAs1DForOutWhenUnconnected=off
  HV_Orientation_BB[x;y;z][rad] : Outport  Port=8  VectorParamsAs1DForOutWhenUnconnected=off
  HV_Current_Curvature[1|m] : Outport  Port=9  VectorParamsAs1DForOutWhenUnconnected=off
  HV_Steering_Angle[rad] : Outport  Port=10  VectorParamsAs1DForOutWhenUnconnected=off
  HV_Steering_Angle_dt[rad|s] : Outport  Port=11  VectorParamsAs1DForOutWhenUnconnected=off
  HV_Steering_Torque[Nm] : Outport  Port=12  VectorParamsAs1DForOutWhenUnconnected=off
  HV_Pos_AccPedal[0_1] : Outport  Port=13  VectorParamsAs1DForOutWhenUnconnected=off
  HV_Pos_ClutchPedal[0_1] : Outport  Port=14  VectorParamsAs1DForOutWhenUnconnected=off
  HV_Gear[] : Outport  Port=15  VectorParamsAs1DForOutWhenUnconnected=off
  HV_Type_Engine[] : Outport  Port=16  VectorParamsAs1DForOutWhenUnconnected=off
  HV_n_Engine[rpm] : Outport  Port=17  VectorParamsAs1DForOutWhenUnconnected=off
  HV_Trq_Engine[Nm] : Outport  Port=18  VectorParamsAs1DForOutWhenUnconnected=off
  HV_Vehicle_Weight[kg] : Outport  Port=19  VectorParamsAs1DForOutWhenUnconnected=off
  HV_Vehicle_Operating_State[] : Outport  Port=20  VectorParamsAs1DForOutWhenUnconnected=off
  HV_WheelData_Axle_Idx[] : Outport  Port=21  VectorParamsAs1DForOutWhenUnconnected=off
  HV_WheelData_Wheel_Idx[] : Outport  Port=22  VectorParamsAs1DForOutWhenUnconnected=off
  HV_WheelData_Wheel_Speed[rad|s] : Outport  Port=23  VectorParamsAs1DForOutWhenUnconnected=off
  HV_WheelData_Wheel_Slip[] : Outport  Port=24  VectorParamsAs1DForOutWhenUnconnected=off
  wires:
  asm_trf_osi_access_host_vehicle_data/24 -> HV_WheelData_Wheel_Slip[]/1
  asm_trf_osi_access_host_vehicle_data/23 -> HV_WheelData_Wheel_Speed[rad|s]/1
  asm_trf_osi_access_host_vehicle_data/22 -> HV_WheelData_Wheel_Idx[]/1
  asm_trf_osi_access_host_vehicle_data/21 -> HV_WheelData_Axle_Idx[]/1
  asm_trf_osi_access_host_vehicle_data/20 -> HV_Vehicle_Operating_State[]/1
  asm_trf_osi_access_host_vehicle_data/19 -> HV_Vehicle_Weight[kg]/1
  asm_trf_osi_access_host_vehicle_data/18 -> HV_Trq_Engine[Nm]/1
  asm_trf_osi_access_host_vehicle_data/17 -> HV_n_Engine[rpm]/1
  asm_trf_osi_access_host_vehicle_data/16 -> HV_Type_Engine[]/1
  asm_trf_osi_access_host_vehicle_data/15 -> HV_Gear[]/1
  asm_trf_osi_access_host_vehicle_data/14 -> HV_Pos_ClutchPedal[0_1]/1
  asm_trf_osi_access_host_vehicle_data/13 -> HV_Pos_AccPedal[0_1]/1
  asm_trf_osi_access_host_vehicle_data/12 -> HV_Steering_Torque[Nm]/1
  asm_trf_osi_access_host_vehicle_data/11 -> HV_Steering_Angle_dt[rad|s]/1
  asm_trf_osi_access_host_vehicle_data/10 -> HV_Steering_Angle[rad]/1
  asm_trf_osi_access_host_vehicle_data/8 -> HV_Orientation_BB[x;y;z][rad]/1
  asm_trf_osi_access_host_vehicle_data/6 -> HV_Velocity_BB[x;y;z][m|s]/1
  asm_trf_osi_access_host_vehicle_data/5 -> HV_Position_BB[x;y;z][m]/1
  asm_trf_osi_access_host_vehicle_data/4 -> HV_Pos_BrakePedal[0_1]/1
  asm_trf_osi_access_host_vehicle_data/3 -> HV_ID[]/1
  asm_trf_osi_access_host_vehicle_data/2 -> Time_Stamp_Nanos[ns]/1
  asm_trf_osi_access_host_vehicle_data/1 -> Time_Stamp_Seconds[s]/1
  Enable[0Off|1On]/1 -> asm_trf_osi_access_host_vehicle_data/1
  OSI_HV_Data/1 -> asm_trf_osi_access_host_vehicle_data/2
  asm_trf_osi_access_host_vehicle_data/9 -> HV_Current_Curvature[1|m]/1
  asm_trf_osi_access_host_vehicle_data/7 -> HV_Acceleration_BB[x;y;z][m|s2]/1

== system ASM_Traffic/Environment/GroundTruth/PlantModel/VehicleBasics/StartButton_Mapping ==
  State_StartButton[-2|-1|0|1|2|3] : Inport
  Multiport Switch1 : MultiPortSwitch  DataPortOrder=Specify indices  DataPortIndices={-2,-1,0,1,2,3}  DataPortForDefault=Additional data port  SaturateOnIntegerOverflow=off  InputSameDT=off
  Operating_State_Driving : Constant  Value=6
  Operating_State_Entertainment : Constant  Value=5
  Operating_State_Other : Constant
  Operating_State_Sleep : Constant  Value=2
  Operating_State_Unknown : Constant  Value=0
  OperatingState[] : Outport
  wires:
  Operating_State_Driving/1 -> Multiport Switch1/7
  Operating_State_Entertainment/1 -> Multiport Switch1/4, Multiport Switch1/5, Multiport Switch1/6
  Multiport Switch1/1 -> OperatingState[]/1
  Operating_State_Other/1 -> Multiport Switch1/2
  Operating_State_Sleep/1 -> Multiport Switch1/3
  State_StartButton[-2|-1|0|1|2|3]/1 -> Multiport Switch1/1
  Operating_State_Unknown/1 -> Multiport Switch1/8

== system ASM_Traffic/Environment/GroundTruth/PlantModel/VehicleLocalization/ChangeLabel ==
  In1 : Inport
  Out1 : Outport  VectorParamsAs1DForOutWhenUnconnected=off
  wires:
  In1/1 -> Out1/1

== system ASM_Traffic/Environment/GroundTruth/UserInterface/DISP_Plant/Interface_Mode[0Off|1ObjOnly|2ObjAndLanes] ==
  In1 : Inport
  Out1 : Outport  VectorParamsAs1DForOutWhenUnconnected=off
  wires:
  In1/1 -> Out1/1

== system ASM_Traffic/Environment/GroundTruth/UserInterface/DISP_Plant/Num_Laneboundaries[] ==
  In1 : Inport
  Out1 : Outport  VectorParamsAs1DForOutWhenUnconnected=off
  wires:
  In1/1 -> Out1/1

== system ASM_Traffic/Environment/GroundTruth/UserInterface/DISP_Plant/Num_Lanes[] ==
  In1 : Inport
  Out1 : Outport  VectorParamsAs1DForOutWhenUnconnected=off
  wires:
  In1/1 -> Out1/1

== system ASM_Traffic/Environment/GroundTruth/UserInterface/DISP_Plant/Num_MovObj[] ==
  In1 : Inport
  Out1 : Outport  VectorParamsAs1DForOutWhenUnconnected=off
  wires:
  In1/1 -> Out1/1

== system ASM_Traffic/Environment/GroundTruth/UserInterface/DISP_Plant/Num_MovObj_in_GT_Area[] ==
  In1 : Inport
  Out1 : Outport  VectorParamsAs1DForOutWhenUnconnected=off
  wires:
  In1/1 -> Out1/1

== system ASM_Traffic/Environment/GroundTruth/UserInterface/DISP_Plant/Num_StatObj[] ==
  In1 : Inport
  Out1 : Outport  VectorParamsAs1DForOutWhenUnconnected=off
  wires:
  In1/1 -> Out1/1

== system ASM_Traffic/Environment/GroundTruth/UserInterface/DISP_Plant/Num_StatObj_in_GT_Area[] ==
  In1 : Inport
  Out1 : Outport  VectorParamsAs1DForOutWhenUnconnected=off
  wires:
  In1/1 -> Out1/1

== system ASM_Traffic/Environment/GroundTruth/UserInterface/DISP_Plant/Num_TrfLights[] ==
  In1 : Inport
  Out1 : Outport  VectorParamsAs1DForOutWhenUnconnected=off
  wires:
  In1/1 -> Out1/1

== system ASM_Traffic/Environment/GroundTruth/UserInterface/DISP_Plant/Num_TrfLights_in_GT_Area[] ==
  In1 : Inport
  Out1 : Outport  VectorParamsAs1DForOutWhenUnconnected=off
  wires:
  In1/1 -> Out1/1

== system ASM_Traffic/Environment/GroundTruth/UserInterface/DISP_Plant/Num_TrfSigns[] ==
  In1 : Inport
  Out1 : Outport  VectorParamsAs1DForOutWhenUnconnected=off
  wires:
  In1/1 -> Out1/1

== system ASM_Traffic/Environment/GroundTruth/UserInterface/DISP_Plant/Num_TrfSigns_in_GT_Area[] ==
  In1 : Inport
  Out1 : Outport  VectorParamsAs1DForOutWhenUnconnected=off
  wires:
  In1/1 -> Out1/1

== system ASM_Traffic/Environment/GroundTruth/UserInterface/PAR_Plant/Ego_Vehicle ==
  Interface_In : Inport
  Brake[] : Constant  Tag=AD:ASM_Sw_SpeedLimit_Source[1Manual|2RoadScenery]  Value=2
  Bus Creator1 : BusCreator  Inputs=3
  Bus Selector : BusSelector  OutputSignals=Maneuver.Plant.UserSignals_Customized.ASM_Vehicle_TurnLights[]
  Ego_Vehicle_Driver_ID[] : Constant  Tag=AD:ASM_Sw_SpeedLimit_Source[1Manual|2RoadScenery]
  Ego_Vehicle_ID[] : Constant  Tag=AD:ASM_Sw_SpeedLimit_Source[1Manual|2RoadScenery]  Value=0
  Emergency_Vehicle_Illumination[] : Constant  Tag=AD:ASM_Sw_SpeedLimit_Source[1Manual|2RoadScenery]  Value=2
  Front_Fog_Light[] : Constant  Tag=AD:ASM_Sw_SpeedLimit_Source[1Manual|2RoadScenery]  Value=2
  Head_Light[] : Constant  Tag=AD:ASM_Sw_SpeedLimit_Source[1Manual|2RoadScenery]  Value=2
  High_Beam[] : Constant  Tag=AD:ASM_Sw_SpeedLimit_Source[1Manual|2RoadScenery]  Value=2
  Indicator_State[] : Subsystem
  License_Plate_Illumination_Rear[] : Constant  Tag=AD:ASM_Sw_SpeedLimit_Source[1Manual|2RoadScenery]  Value=2
  Mux : Mux  Inputs=10
  Rear_Fog_Light[] : Constant  Tag=AD:ASM_Sw_SpeedLimit_Source[1Manual|2RoadScenery]  Value=2
  Reversing_Light[] : Constant  Tag=AD:ASM_Sw_SpeedLimit_Source[1Manual|2RoadScenery]  Value=2
  Service_Vehicle_Illumination[] : Constant  Tag=AD:ASM_Sw_SpeedLimit_Source[1Manual|2RoadScenery]  Value=2
  Ego_Vehicle[] : Outport  VectorParamsAs1DForOutWhenUnconnected=off
  wires:
  Bus Selector/1 -> Indicator_State[]/1(ASM_Vehicle_TurnLights[])  "<ASM_Vehicle_TurnLights[]>"
  Reversing_Light[]/1 -> Mux/2
  High_Beam[]/1 -> Mux/1
  Front_Fog_Light[]/1 -> Mux/3
  Bus Creator1/1 -> Ego_Vehicle[]/1  "Ego_Vehicle[]"
  License_Plate_Illumination_Rear[]/1 -> Mux/5
  Indicator_State[]/1(Indicator_State[]) -> Mux/9
  Brake[]/1 -> Mux/10
  Rear_Fog_Light[]/1 -> Mux/6
  Ego_Vehicle_Driver_ID[]/1 -> Bus Creator1/2  "Ego_Vehicle_Driver_ID[]"
  Mux/1 -> Bus Creator1/3  "Ego_Vehicle_LightStates[]"
  Ego_Vehicle_ID[]/1 -> Bus Creator1/1  "Ego_Vehicle_ID[]"
  Head_Light[]/1 -> Mux/4
  Emergency_Vehicle_Illumination[]/1 -> Mux/7
  Service_Vehicle_Illumination[]/1 -> Mux/8
  Interface_In/1 -> Bus Selector/1

== system ASM_Traffic/Environment/GroundTruth/UserInterface/PAR_Plant/Environmental_Conditions ==
  Add : Sum
  Ambient_Illumination[] : Constant  Tag=AD:ASM_Sw_SpeedLimit_Source[1Manual|2RoadScenery]
  Atmospheric_Pressure[Pa] : Constant  Tag=AD:ASM_Sw_SpeedLimit_Source[1Manual|2RoadScenery]  Value=101325
  Constant1 : Constant  Value=86400
  EnvConditions_Fog[] : Constant  Tag=AD:ASM_Sw_SpeedLimit_Source[1Manual|2RoadScenery]
  Gain : Gain  Gain=3600
  Math Function : Math  Operator=rem  SignedPower=on
  Mux : Mux  Inputs=8
  Precipitation[] : Constant  Tag=AD:ASM_Sw_SpeedLimit_Source[1Manual|2RoadScenery]
  Relative_Humidity[%] : Constant  Tag=AD:ASM_Sw_SpeedLimit_Source[1Manual|2RoadScenery]
  Start_Unix_Timestamp[s] : Constant  Tag=AD:ASM_Sw_SpeedLimit_Source[1Manual|2RoadScenery]  Value=1588809600
  Temperature[K] : Constant  Tag=AD:ASM_Sw_SpeedLimit_Source[1Manual|2RoadScenery]  Value=290
  UTC_Offset[h] : Constant  Tag=AD:ASM_Sw_SpeedLimit_Source[1Manual|2RoadScenery]  Value=2
  Environmental_Conditions[] : Outport  VectorParamsAs1DForOutWhenUnconnected=off
  wires:
  Mux/1 -> Environmental_Conditions[]/1  "Environmental_Conditions[]"
  Ambient_Illumination[]/1 -> Mux/2  "Ambient_Illumination[]"
  Precipitation[]/1 -> Mux/1  "Precipitation[]"
  Temperature[K]/1 -> Mux/4  "Temperature[K]"
  Relative_Humidity[%]/1 -> Mux/5  "Relative_Humidity[%]"
  EnvConditions_Fog[]/1 -> Mux/3  "EnvConditions_Fog[]"
  Atmospheric_Pressure[Pa]/1 -> Mux/6  "Atmospheric_Pressure[Pa]"
  Start_Unix_Timestamp[s]/1 -> Add/2, Mux/8  "Start_Unix_Timestamp[s]"
  Constant1/1 -> Math Function/2
  UTC_Offset[h]/1 -> Gain/1
  Gain/1 -> Add/1
  Math Function/1 -> Mux/7  "Start_Seconds_Since_Midnight[s]"
  Add/1 -> Math Function/1
